simulink model "s_b4a4x4kf"  (R2018a)
settings: Solver=VariableStepDiscrete  StartTime=0.0  StopTime=1  RelTol=1e-3
undefined symbols (not defined in the file): fft_stages, n_bits_ants, n_bits_xengs
libraries: xbsIndex_r4 x22457, casper_library_misc x31, xbsReplacements_r4 x30, casper_library_scopes x17, xps_library x4
(part 155 of 232)

== system s_b4a4x4kf/sys0/vacc/vacc_time/snap/buscreate ==
  in1 : Inport
  in2 : Inport  Port=2
  in3 : Inport  Port=3
  in4 : Inport  Port=4
  in5 : Inport  Port=5
  in6 : Inport  Port=6
  in7 : Inport  Port=7
  in8 : Inport  Port=8
  in9 : Inport  Port=9
  in10 : Inport  Port=10
  concatenate : xbsIndex_r4/Concat  num_inputs=10  dbl_ovrd=off  block_type=concat
  reinterpret{1..10} (10 alike) : xbsIndex_r4/Reinterpret  force_arith_type=on  arith_type=Unsigned  force_bin_pt=on  bin_pt=0  block_type=reinterpret
      reinterpret1 settings: infoedit="Changes signal type without altering the binary representation.   You can changed the signal between signed and unsigned, and relocate the binary point.<br><br>Hardware notes: In hardware this block costs nothing.<br><br>Example:  Suppose the input is 6 bits wide, signed, with 2 fractional bits, and the output is forced to unsigned with 0 fractional bits.  Then an input of -2.0 (1110.00 in binary 2's complement) becomes an output of 56 (111000 in binary)."
      reinterpret2 settings: infoedit="Changes signal type without altering the binary representation.   You can changed the signal between signed and unsigned, and relocate the binary point.<br><br>Hardware notes: In hardware this block costs nothing.<br><br>Example:  Suppose the input is 6 bits wide, signed, with 2 fractional bits, and the output is forced to unsigned with 0 fractional bits.  Then an input of -2.0 (1110.00 in binary 2's complement) becomes an output of 56 (111000 in binary)."
  bus_out : Outport
  wires:
  concatenate/1 -> bus_out/1
  in1/1 -> reinterpret1/1
  reinterpret1/1 -> concatenate/1
  in2/1 -> reinterpret2/1
  reinterpret2/1 -> concatenate/2
  in3/1 -> reinterpret3/1
  reinterpret3/1 -> concatenate/3
  in4/1 -> reinterpret4/1
  reinterpret4/1 -> concatenate/4
  in5/1 -> reinterpret5/1
  reinterpret5/1 -> concatenate/5
  in6/1 -> reinterpret6/1
  reinterpret6/1 -> concatenate/6
  in7/1 -> reinterpret7/1
  reinterpret7/1 -> concatenate/7
  in8/1 -> reinterpret8/1
  reinterpret8/1 -> concatenate/8
  in9/1 -> reinterpret9/1
  reinterpret9/1 -> concatenate/9
  in10/1 -> reinterpret10/1
  reinterpret10/1 -> concatenate/10

== system s_b4a4x4kf/sys0/vacc/vacc_time/snap/io_delay ==
  d : Inport
  Register0 : xbsIndex_r4/Register  init=0  rst=off  en=off  dbl_ovrd=off  block_type=register
      settings: block_version=11.4
  Register1 : xbsIndex_r4/Register  init=0  rst=off  en=off  dbl_ovrd=off  block_type=register
      settings: block_version=11.4
  q : Outport
  wires:
  Register1/1 -> q/1
  d/1 -> Register0/1
  Register0/1 -> Register1/1

== system s_b4a4x4kf/sys0/vacc/vacc_time/snap/ss ==
  note: Generate stop
      | when in circular
      | capture mode
  note: Delay start
      | of capture
  note: ctrl:
      | bit0: Put a posedge here
      |         to enable a new capture.
      | bit1: ignore external trigger
      |         and trigger immediately.
      | bit2: ignore external write
      |         enable and capture on
      |         every FPGA clock.
      | bit3: continuously capture
      |         data until we get an
      |         external stop command.
  note: Offset in vector
      | from first element
      | captured, used
      | during circular capture
  note: Number of
      | bytes in
      | buffer and
      | done bit
  note: Number of valid
      | data samples to
      | skip after trigger
      | before starting
      | capture
  note: Value on vin
      | aligned with
      | first sample on
      | din captured
  din : Inport
  we : Inport  Port=2
  trig : Inport  Port=3
  stop : Inport  Port=4
  add_del : xbsIndex_r4/Delay  rst=off  infoeditControl=Selection of Reset will increase slice count due to use of real FFs and instead of SRLs  en=off  latency=1  reg_retiming=on  dbl_ovrd=off  block_type=delay
      settings: block_version=11.4
  add_gen : Subsystem  AncestorBlock=casper_library_scopes/snapshot/add_gen  mask{counter_size=32, increment=8, nsamples=11, burst_size=0, use_dsp48=on}
      mask prompts: counter_size "Address counter size (2^?)"; increment "Address counter increment"; nsamples "Number of samples (2^?)"; burst_size "Burst size (2^?)"; use_dsp48 "dsp48 counter/s"
      mask init:
      | set_param(gcb,'LinkStatus','inactive');
      | if strcmp(use_dsp48,'on'),
      |     set_param([gcb,'/add_gen'],'implementation','DSP48');
      | else
      |     set_param([gcb,'/add_gen'],'implementation','Fabric');
      | end
  arm : xbsIndex_r4/Constant  const=0  gui_display_data_type=Fixed-point  arith_type=Boolean  n_bits=16  bin_pt=14  preci_type=Single  exp_width=8  frac_width=24  explicit_period=on  period=1  equ=P=C  opselect=C  inp2=PCIN>>17  opr=+  inp1=P  carry=CIN  dbl_ovrd=off  block_type=constant
  arm_or : xbsIndex_r4/Logical  logical_function=OR  inputs=2  en=off  latency=0  precision=Full  arith_type=Unsigned  n_bits=16  bin_pt=0  align_bp=on  dbl_ovrd=off  block_type=logical
  basic_ctrl : Subsystem  AncestorBlock=casper_library_scopes/snapshot/basic_ctrl  mask{dram=off, data_width=64}
      mask prompts: data_width "data width"
      mask init:
      | set_param(gcb,'LinkStatus','inactive');
      | set_param([gcb,'/dram_munge'], 'dram', dram);
  bram : Subsystem  Tag=xps:bram  AncestorBlock=xps_library/Memory/shared_bram  mask{arith_type=Unsigned, addr_width=11, data_width=64, reg_prim_output=off, reg_core_output=off, optimization=Minimum_Area, data_bin_pt=0, init_vals=[0:2^11-1], sample_rate=1}
      mask prompts: arith_type "Output Data Type"; addr_width "Address width"; data_width "Data Width"; reg_prim_output "Register Primitive Output"; reg_core_output "Register Core Output"; data_bin_pt "Data Binary Point"; init_vals "Initial values (simulation only)"; sample_rate "Sample rate"
      mask init:
      | shared_bram_mask;
      mask TypeOptions arith_type: Unsigned | Signed  (2's comp)
      mask TypeOptions data_width: 8 | 16 | 32 | 64 | 128
      mask TypeOptions optimization: Minimum_Area | Low_Power
  cast : xbsIndex_r4/Convert  gui_display_data_type=Fixed-point  arith_type=Unsigned  n_bits=64  bin_pt=0  float_type=Single  exp_bits=8  fraction_bits=24  quantization=Truncate  overflow=Wrap  en=off  latency=0  pipeline=off  dbl_ovrd=off  block_type=convert
      settings: block_version=11.4
  circ : xbsIndex_r4/Constant  const=0  gui_display_data_type=Fixed-point  arith_type=Boolean  n_bits=16  bin_pt=14  preci_type=Single  exp_width=8  frac_width=24  explicit_period=on  period=1  equ=P=C  opselect=C  inp2=PCIN>>17  opr=+  inp1=P  carry=CIN  dbl_ovrd=off  block_type=constant
  circ_or : xbsIndex_r4/Logical  logical_function=OR  inputs=2  en=off  latency=0  precision=Full  arith_type=Unsigned  n_bits=16  bin_pt=0  align_bp=on  dbl_ovrd=off  block_type=logical
  ctrl : Subsystem  Tag=xps:sw_reg  AncestorBlock=xps_library/Memory/software_register  mask(swreg){io_dir=From Processor, io_delay=0, init_val=0, sample_period=1, names=reg, bitwidths=32, bin_pts=0, arith_types=0, sim_port=off, show_format=on}
      mask prompts: io_dir "I/O direction"; io_delay "I/O delay"; init_val "Initial Value"; sample_period "Sample period"; names "Bitfield names [msb...lsb]"; bitwidths "Bitfield widths"; bin_pts "Bitfield binary pts"; arith_types "Bitfield types, ufix=0, fix=1, bool=2"; sim_port "Provide sim input/output?"; show_format "Print format string?"
      mask help: A 32-bit software-accessible register. Can be divided into bitfields of varying widths and types using the fields in the block mask.
      mask init:
      | swreg_init(gcb)
      settings: AttributesFormatString=1input:uf32.0 = 32 bits
      mask TypeOptions io_dir: To Processor | From Processor
      mask Callback io_dir:
      | mask_enables = get_param(gcb, 'MaskEnables');
      | mask_names = get_param(gcb, 'MaskNames');
      | if strcmp(get_param(gcb, 'io_dir'), 'To Processor'),
      |     mask_enables{ismember(mask_names, 'sample_period')} = 'off';
      | else
      |     mask_enables{ismember(mask_names, 'sample_period')} = 'on';
      | end
      | set_param(gcb, 'MaskEnables', mask_enables);
      mask DialogControl ParameterTabVar0 Prompt: Setup
  ctrl_combine : Subsystem  AncestorBlock=casper_library_flow_control/bus_create  mask(bus_create){inputNum=4}
      mask prompts: inputNum "Number of inputs:"
      mask init:
      | bus_create_init(gcb,...
      |     'inputNum', inputNum);
  ctrl_split : Subsystem  AncestorBlock=casper_library_flow_control/bus_expand  mask(bus_expand){mode=divisions of arbitrary size, outputNum=1, outputWidth=[28 1 2 1], outputBinaryPt=0, outputArithmeticType=[0 2 0 2], show_format=on, outputToWorkspace=off, variablePrefix=out, outputToModelAsWell=on}
      mask prompts: outputNum "Number of outputs:"; outputWidth "Output width [msb ... lsb]:"; outputBinaryPt "Output binary point position [msb ... lsb]:"; outputArithmeticType "Output arithmetic type (ufix=0, fix=1, bool=2) [msb ... lsb]:"; show_format "Print format string?"; outputToWorkspace "Output to workspace?"; variablePrefix "Variable name prefix:"; outputToModelAsWell "Output to model as well?"
      mask help:
      | Expands a 'bus' made using a bus_create or Xilinx
      | concat block.
      | The input will be divided into the specified number
      | of outputs with the specified arithmetic types.
      | Divisions are made from most significant bit.
      mask init: same as s_b4a4x4kf/bus_expand
      settings: AttributesFormatString=4 outputs: uf28.0,b,uf2.0,b,
      mask TypeOptions mode: divisions of equal size | divisions of arbitrary size
      mask Callback mode: bus_expand_callback();
      mask Callback outputWidth: bus_expand_callback();
      mask Callback outputToWorkspace: bus_expand_callback();
  dat_del : xbsIndex_r4/Delay  rst=off  infoeditControl=Selection of Reset will increase slice count due to use of real FFs and instead of SRLs  en=off  latency=1  reg_retiming=on  dbl_ovrd=off  block_type=delay
      settings: block_version=11.4
  gbram : Terminator
  goto_ss_we2_const : xbsIndex_r4/Constant  const=0  gui_display_data_type=Fixed-point  arith_type=Boolean  n_bits=16  bin_pt=14  preci_type=Single  exp_width=8  frac_width=24  explicit_period=on  period=1  equ=P=C  opselect=C  inp2=PCIN>>17  opr=+  inp1=P  carry=CIN  dbl_ovrd=off  block_type=constant
  gval : Terminator
  ri : xbsIndex_r4/Reinterpret  force_arith_type=on  arith_type=Unsigned  force_bin_pt=on  bin_pt=0  block_type=reinterpret
      settings: infoedit="Changes signal type without altering the binary representation.   You can changed the signal between signed and unsigned, and relocate the binary point.<br><br>Hardware notes: In hardware this block costs nothing.<br><br>Example:  Suppose the input is 6 bits wide, signed, with 2 fractional bits, and the output is forced to unsigned with 0 fractional bits.  Then an input of -2.0 (1110.00 in binary 2's complement) becomes an output of 56 (111000 in binary)."
  status : Subsystem  Tag=xps:sw_reg  AncestorBlock=xps_library/Memory/software_register  mask(swreg){io_dir=To Processor, io_delay=0, init_val=0, sample_period=1, names=reg, bitwidths=32, bin_pts=0, arith_types=0, sim_port=off, show_format=on}
      mask prompts: io_dir "I/O direction"; io_delay "I/O delay"; init_val "Initial Value"; sample_period "Sample period"; names "Bitfield names [msb...lsb]"; bitwidths "Bitfield widths"; bin_pts "Bitfield binary pts"; arith_types "Bitfield types, ufix=0, fix=1, bool=2"; sim_port "Provide sim input/output?"; show_format "Print format string?"
      mask help: A 32-bit software-accessible register. Can be divided into bitfields of varying widths and types using the fields in the block mask.
      mask init:
      | swreg_init(gcb)
      settings: AttributesFormatString=1output:uf32.0 = 32 bits
      mask TypeOptions io_dir: To Processor | From Processor
      mask Callback io_dir:
      | mask_enables = get_param(gcb, 'MaskEnables');
      | mask_names = get_param(gcb, 'MaskNames');
      | if strcmp(get_param(gcb, 'io_dir'), 'To Processor'),
      |     mask_enables{ismember(mask_names, 'sample_period')} = 'off';
      | else
      |     mask_enables{ismember(mask_names, 'sample_period')} = 'on';
      | end
      | set_param(gcb, 'MaskEnables', mask_enables);
      mask DialogControl ParameterTabVar0 Prompt: Setup
  stop_gen : casper_library_scopes/snapshot/stop_gen
      settings: SourceProductName=CASPER DSP Blockset
  tr_en_cnt : Subsystem  Tag=xps:sw_reg  AncestorBlock=xps_library/Memory/software_register  mask(swreg){io_dir=To Processor, io_delay=0, init_val=0, sample_period=1, names=reg, bitwidths=32, bin_pts=0, arith_types=0, sim_port=off, show_format=on}
      mask prompts: io_dir "I/O direction"; io_delay "I/O delay"; init_val "Initial Value"; sample_period "Sample period"; names "Bitfield names [msb...lsb]"; bitwidths "Bitfield widths"; bin_pts "Bitfield binary pts"; arith_types "Bitfield types, ufix=0, fix=1, bool=2"; sim_port "Provide sim input/output?"; show_format "Print format string?"
      mask help: A 32-bit software-accessible register. Can be divided into bitfields of varying widths and types using the fields in the block mask.
      mask init:
      | swreg_init(gcb)
      settings: AttributesFormatString=1output:uf32.0 = 32 bits
      mask TypeOptions io_dir: To Processor | From Processor
      mask Callback io_dir:
      | mask_enables = get_param(gcb, 'MaskEnables');
      | mask_names = get_param(gcb, 'MaskNames');
      | if strcmp(get_param(gcb, 'io_dir'), 'To Processor'),
      |     mask_enables{ismember(mask_names, 'sample_period')} = 'off';
      | else
      |     mask_enables{ismember(mask_names, 'sample_period')} = 'on';
      | end
      | set_param(gcb, 'MaskEnables', mask_enables);
      mask DialogControl ParameterTabVar0 Prompt: Setup
  vin_const : xbsIndex_r4/Constant  const=0  gui_display_data_type=Fixed-point  arith_type=Boolean  n_bits=16  bin_pt=14  preci_type=Single  exp_width=8  frac_width=24  explicit_period=on  period=1  equ=P=C  opselect=C  inp2=PCIN>>17  opr=+  inp1=P  carry=CIN  dbl_ovrd=off  block_type=constant
  we_del : xbsIndex_r4/Delay  rst=off  infoeditControl=Selection of Reset will increase slice count due to use of real FFs and instead of SRLs  en=off  latency=1  reg_retiming=on  dbl_ovrd=off  block_type=delay
      settings: block_version=11.4
  arm_out : Outport
  tag scope: goto_98869994_we1=global, goto_98869994_we2=global, goto_98869994_we3=global, goto_98869994_we4=global
  wires:
  din/1 -> ri/1
  ri/1 -> cast/1
  cast/1 -> basic_ctrl/2(din)
  we/1 -> basic_ctrl/3(we)
  trig/1 -> basic_ctrl/4(trig)
  ctrl_combine/1(bus_out) -> basic_ctrl/5(ctrl), stop_gen/7
  stop/1 -> basic_ctrl/6(stopi)
  arm/1 -> arm_or/2
  arm_or/1 -> arm_out/1, ctrl_combine/4(in4)
  circ/1 -> circ_or/2
  ctrl/1(in_reg) -> ctrl_split/1(bus_in)
  ctrl_split/1(msb_out4) -> ctrl_combine/1(in1)
  ctrl_split/2(out3) -> circ_or/1
  ctrl_split/3(out2) -> ctrl_combine/3(in3)
  ctrl_split/4(lsb_out1) -> arm_or/1
  circ_or/1 -> ctrl_combine/2(in2)
  basic_ctrl/1(vout) -> stop_gen/1
  basic_ctrl/2(dout) -> stop_gen/2
  basic_ctrl/3(we_o) -> stop_gen/3, [goto_98869994_we1]
  basic_ctrl/4(go) -> stop_gen/4
  basic_ctrl/5(stop) -> stop_gen/5
  basic_ctrl/6(init) -> stop_gen/6
  stop_gen/1 -> add_gen/1(vin)
  stop_gen/2 -> add_gen/2(din)
  stop_gen/3 -> add_gen/3(we), [goto_98869994_we3]
  stop_gen/4 -> add_gen/4(go)
  stop_gen/5 -> add_gen/5(cont)
  stop_gen/6 -> add_gen/6(init)
  add_gen/5(status) -> status/1(out_reg)
  vin_const/1 -> basic_ctrl/1(vin)
  add_gen/1(vout) -> gval/1
  add_gen/6(en_cnt) -> tr_en_cnt/1(out_reg)
  add_gen/2(add) -> add_del/1
  add_gen/3(dout) -> dat_del/1
  add_gen/4(we_o) -> we_del/1, [goto_98869994_we4]
  add_del/1 -> bram/1(addr)
  dat_del/1 -> bram/2(data_in)
  we_del/1 -> bram/3(we)
  bram/1(data_out) -> gbram/1
  goto_ss_we2_const/1 -> [goto_98869994_we2]

== system s_b4a4x4kf/sys0/vacc/vacc_time/snap/stop_delay ==
  d : Inport
  Register0 : xbsIndex_r4/Register  init=0  rst=off  en=off  dbl_ovrd=off  block_type=register
      settings: block_version=11.4
  Register1 : xbsIndex_r4/Register  init=0  rst=off  en=off  dbl_ovrd=off  block_type=register
      settings: block_version=11.4
  q : Outport
  wires:
  Register1/1 -> q/1
  d/1 -> Register0/1
  Register0/1 -> Register1/1

== system s_b4a4x4kf/sys0/vacc/vacc_time/snap/trig_delay ==
  d : Inport
  Register0 : xbsIndex_r4/Register  init=0  rst=off  en=off  dbl_ovrd=off  block_type=register
      settings: block_version=11.4
  Register1 : xbsIndex_r4/Register  init=0  rst=off  en=off  dbl_ovrd=off  block_type=register
      settings: block_version=11.4
  q : Outport
  wires:
  Register1/1 -> q/1
  d/1 -> Register0/1
  Register0/1 -> Register1/1

== system s_b4a4x4kf/sys0/vacc/vacc_time/snap/we_delay ==
  d : Inport
  Register0 : xbsIndex_r4/Register  init=0  rst=off  en=off  dbl_ovrd=off  block_type=register
      settings: block_version=11.4
  Register1 : xbsIndex_r4/Register  init=0  rst=off  en=off  dbl_ovrd=off  block_type=register
      settings: block_version=11.4
  q : Outport
  wires:
  Register1/1 -> q/1
  d/1 -> Register0/1
  Register0/1 -> Register1/1

== system s_b4a4x4kf/sys0/vacc_tvg0/generate_time/segment/edge_detect ==
  in : Inport
  Delay : xbsIndex_r4/Delay  rst=off  infoeditControl=Selection of Reset will increase slice count due to use of real FFs and instead of SRLs  en=off  latency=1  reg_retiming=off  dbl_ovrd=off  block_type=delay
      settings: xl_area=[0, 0, 0, 0, 0, 0, 0]
  Inverter : xbsIndex_r4/Inverter  en=off  latency=0  dbl_ovrd=off  block_type=inv
      settings: xl_area=[0, 0, 0, 0, 0, 0, 0]
  edge_op : xbsIndex_r4/Logical  logical_function=NOR  inputs=2  en=off  latency=0  precision=Full  arith_type=Unsigned  n_bits=8  bin_pt=2  align_bp=on  dbl_ovrd=off  block_type=logical
      settings: xl_area=[0, 0, 0, 0, 0, 0, 0]
  out : Outport
  wires:
  Inverter/1 -> edge_op/1
  edge_op/1 -> out/1
  in/1 -> Inverter/1, Delay/1
  Delay/1 -> edge_op/2

== system s_b4a4x4kf/sys0/vacc_tvg0/ins_counter/bus_replicate1/bussify ==
  in1 : Inport
  in2 : Inport  Port=2
  in3 : Inport  Port=3
  in4 : Inport  Port=4
  in5 : Inport  Port=5
  in6 : Inport  Port=6
  in7 : Inport  Port=7
  in8 : Inport  Port=8
  concatenate : xbsIndex_r4/Concat  num_inputs=8  dbl_ovrd=off  block_type=concat
  reinterpret{1..8} (8 alike) : xbsIndex_r4/Reinterpret  force_arith_type=on  arith_type=Unsigned  force_bin_pt=on  bin_pt=0  block_type=reinterpret
      reinterpret1 settings: infoedit="Changes signal type without altering the binary representation.   You can changed the signal between signed and unsigned, and relocate the binary point.<br><br>Hardware notes: In hardware this block costs nothing.<br><br>Example:  Suppose the input is 6 bits wide, signed, with 2 fractional bits, and the output is forced to unsigned with 0 fractional bits.  Then an input of -2.0 (1110.00 in binary 2's complement) becomes an output of 56 (111000 in binary)."
      reinterpret2 settings: infoedit="Changes signal type without altering the binary representation.   You can changed the signal between signed and unsigned, and relocate the binary point.<br><br>Hardware notes: In hardware this block costs nothing.<br><br>Example:  Suppose the input is 6 bits wide, signed, with 2 fractional bits, and the output is forced to unsigned with 0 fractional bits.  Then an input of -2.0 (1110.00 in binary 2's complement) becomes an output of 56 (111000 in binary)."
  bus_out : Outport
  wires:
  concatenate/1 -> bus_out/1
  in1/1 -> reinterpret1/1
  reinterpret1/1 -> concatenate/1
  in2/1 -> reinterpret2/1
  reinterpret2/1 -> concatenate/2
  in3/1 -> reinterpret3/1
  reinterpret3/1 -> concatenate/3
  in4/1 -> reinterpret4/1
  reinterpret4/1 -> concatenate/4
  in5/1 -> reinterpret5/1
  reinterpret5/1 -> concatenate/5
  in6/1 -> reinterpret6/1
  reinterpret6/1 -> concatenate/6
  in7/1 -> reinterpret7/1
  reinterpret7/1 -> concatenate/7
  in8/1 -> reinterpret8/1
  reinterpret8/1 -> concatenate/8

== system s_b4a4x4kf/sys0/vacc_tvg0/ins_counter2/bus_replicate1/bussify ==
  in1 : Inport
  in2 : Inport  Port=2
  in3 : Inport  Port=3
  in4 : Inport  Port=4
  in5 : Inport  Port=5
  in6 : Inport  Port=6
  in7 : Inport  Port=7
  in8 : Inport  Port=8
  concatenate : xbsIndex_r4/Concat  num_inputs=8  dbl_ovrd=off  block_type=concat
  reinterpret{1..8} (8 alike) : xbsIndex_r4/Reinterpret  force_arith_type=on  arith_type=Unsigned  force_bin_pt=on  bin_pt=0  block_type=reinterpret
      reinterpret1 settings: infoedit="Changes signal type without altering the binary representation.   You can changed the signal between signed and unsigned, and relocate the binary point.<br><br>Hardware notes: In hardware this block costs nothing.<br><br>Example:  Suppose the input is 6 bits wide, signed, with 2 fractional bits, and the output is forced to unsigned with 0 fractional bits.  Then an input of -2.0 (1110.00 in binary 2's complement) becomes an output of 56 (111000 in binary)."
      reinterpret2 settings: infoedit="Changes signal type without altering the binary representation.   You can changed the signal between signed and unsigned, and relocate the binary point.<br><br>Hardware notes: In hardware this block costs nothing.<br><br>Example:  Suppose the input is 6 bits wide, signed, with 2 fractional bits, and the output is forced to unsigned with 0 fractional bits.  Then an input of -2.0 (1110.00 in binary 2's complement) becomes an output of 56 (111000 in binary)."
  bus_out : Outport
  wires:
  concatenate/1 -> bus_out/1
  in1/1 -> reinterpret1/1
  reinterpret1/1 -> concatenate/1
  in2/1 -> reinterpret2/1
  reinterpret2/1 -> concatenate/2
  in3/1 -> reinterpret3/1
  reinterpret3/1 -> concatenate/3
  in4/1 -> reinterpret4/1
  reinterpret4/1 -> concatenate/4
  in5/1 -> reinterpret5/1
  reinterpret5/1 -> concatenate/5
  in6/1 -> reinterpret6/1
  reinterpret6/1 -> concatenate/6
  in7/1 -> reinterpret7/1
  reinterpret7/1 -> concatenate/7
  in8/1 -> reinterpret8/1
  reinterpret8/1 -> concatenate/8

== system s_b4a4x4kf/sys0/vacc_tvg0/ins_counter2/segment/edge_detect ==
  in : Inport
  Delay : xbsIndex_r4/Delay  rst=off  infoeditControl=Selection of Reset will increase slice count due to use of real FFs and instead of SRLs  en=off  latency=1  reg_retiming=off  dbl_ovrd=off  block_type=delay
      settings: xl_area=[0, 0, 0, 0, 0, 0, 0]
  Inverter : xbsIndex_r4/Inverter  en=off  latency=0  dbl_ovrd=off  block_type=inv
      settings: xl_area=[0, 0, 0, 0, 0, 0, 0]
  edge_op : xbsIndex_r4/Logical  logical_function=NOR  inputs=2  en=off  latency=0  precision=Full  arith_type=Unsigned  n_bits=8  bin_pt=2  align_bp=on  dbl_ovrd=off  block_type=logical
      settings: xl_area=[0, 0, 0, 0, 0, 0, 0]
  out : Outport
  wires:
  Inverter/1 -> edge_op/1
  edge_op/1 -> out/1
  in/1 -> Inverter/1, Delay/1
  Delay/1 -> edge_op/2

== system s_b4a4x4kf/sys0/vacc_tvg0/ins_counter3/bus_replicate1/bussify ==
  in1 : Inport
  in2 : Inport  Port=2
  in3 : Inport  Port=3
  in4 : Inport  Port=4
  in5 : Inport  Port=5
  in6 : Inport  Port=6
  in7 : Inport  Port=7
  in8 : Inport  Port=8
  concatenate : xbsIndex_r4/Concat  num_inputs=8  dbl_ovrd=off  block_type=concat
  reinterpret{1..8} (8 alike) : xbsIndex_r4/Reinterpret  force_arith_type=on  arith_type=Unsigned  force_bin_pt=on  bin_pt=0  block_type=reinterpret
      reinterpret1 settings: infoedit="Changes signal type without altering the binary representation.   You can changed the signal between signed and unsigned, and relocate the binary point.<br><br>Hardware notes: In hardware this block costs nothing.<br><br>Example:  Suppose the input is 6 bits wide, signed, with 2 fractional bits, and the output is forced to unsigned with 0 fractional bits.  Then an input of -2.0 (1110.00 in binary 2's complement) becomes an output of 56 (111000 in binary)."
      reinterpret2 settings: infoedit="Changes signal type without altering the binary representation.   You can changed the signal between signed and unsigned, and relocate the binary point.<br><br>Hardware notes: In hardware this block costs nothing.<br><br>Example:  Suppose the input is 6 bits wide, signed, with 2 fractional bits, and the output is forced to unsigned with 0 fractional bits.  Then an input of -2.0 (1110.00 in binary 2's complement) becomes an output of 56 (111000 in binary)."
  bus_out : Outport
  wires:
  concatenate/1 -> bus_out/1
  in1/1 -> reinterpret1/1
  reinterpret1/1 -> concatenate/1
  in2/1 -> reinterpret2/1
  reinterpret2/1 -> concatenate/2
  in3/1 -> reinterpret3/1
  reinterpret3/1 -> concatenate/3
  in4/1 -> reinterpret4/1
  reinterpret4/1 -> concatenate/4
  in5/1 -> reinterpret5/1
  reinterpret5/1 -> concatenate/5
  in6/1 -> reinterpret6/1
  reinterpret6/1 -> concatenate/6
  in7/1 -> reinterpret7/1
  reinterpret7/1 -> concatenate/7
  in8/1 -> reinterpret8/1
  reinterpret8/1 -> concatenate/8

== system s_b4a4x4kf/sys0/vacc_tvg0/ins_counter3/segment/edge_detect ==
  in : Inport
  Delay : xbsIndex_r4/Delay  rst=off  infoeditControl=Selection of Reset will increase slice count due to use of real FFs and instead of SRLs  en=off  latency=1  reg_retiming=off  dbl_ovrd=off  block_type=delay
      settings: xl_area=[0, 0, 0, 0, 0, 0, 0]
  Inverter : xbsIndex_r4/Inverter  en=off  latency=0  dbl_ovrd=off  block_type=inv
      settings: xl_area=[0, 0, 0, 0, 0, 0, 0]
  edge_op : xbsIndex_r4/Logical  logical_function=NOR  inputs=2  en=off  latency=0  precision=Full  arith_type=Unsigned  n_bits=8  bin_pt=2  align_bp=on  dbl_ovrd=off  block_type=logical
      settings: xl_area=[0, 0, 0, 0, 0, 0, 0]
  out : Outport
  wires:
  Inverter/1 -> edge_op/1
  edge_op/1 -> out/1
  in/1 -> Inverter/1, Delay/1
  Delay/1 -> edge_op/2

== system s_b4a4x4kf/sys0/xeng/auto_tap/dual_pol_cmac/cmac1 ==
  a+bi : Inport
  c+di : Inport  Port=2
  acc_in : Inport  Port=3
  sync : Inport  Port=4
  valid_in : Inport  Port=5
  Constant1 : xbsIndex_r4/Constant  const=0  gui_display_data_type=Fixed-point  arith_type=Unsigned  n_bits=bit_growth  bin_pt=0  preci_type=Single  exp_width=8  frac_width=24  explicit_period=on  period=1  equ=P=C  opselect=C  inp2=PCIN>>17  opr=+  inp1=P  carry=CIN  dbl_ovrd=off  block_type=constant
      settings: block_version=9.2.01
  Constant2 : xbsIndex_r4/Constant  const=0  gui_display_data_type=Fixed-point  arith_type=Unsigned  n_bits=1  bin_pt=0  preci_type=Single  exp_width=8  frac_width=24  explicit_period=off  period=1  equ=P=C  opselect=C  inp2=PCIN>>17  opr=+  inp1=P  carry=CIN  dbl_ovrd=off  block_type=constant
      settings: block_version=9.2.01
  Counter : xbsIndex_r4/Counter  cnt_type=Count Limited  cnt_to=acc_len - 1  operation=Up  start_count=0  cnt_by_val=1  arith_type=Unsigned  n_bits=bit_growth  bin_pt=0  load_pin=off  rst=on  en=off  explicit_period=off  period=1  use_behavioral_HDL=off  implementation=Fabric  use_rpm=on  dbl_ovrd=off  block_type=counter
      settings: xl_area=[0, 0, 0, 0, 0, 0, 0]  block_version=9.2.01
  Delay : xbsIndex_r4/Delay  rst=off  infoeditControl=Selection of Reset will increase slice count due to use of real FFs and instead of SRLs  en=off  latency=add_latency + mult_latency - 1  reg_retiming=on  dbl_ovrd=off  block_type=delay
      settings: xl_area=[0, 0, 0, 0, 0, 0, 0]  block_version=9.2.01
  Relational : xbsIndex_r4/Relational  mode=a=b  op_type=Bool  en=off  latency=1  dbl_ovrd=off  block_type=relational
      settings: xl_area=[0, 0, 0, 0, 0, 0, 0]  block_version=9.2.01
  Terminator : Terminator
  acc : Subsystem
  acc1 : Subsystem
  c_to_ri1 : Subsystem
  c_to_ri2 : Subsystem
  cmult* : Subsystem  mask(cmult){n_bits_a=8, bin_pt_a=7, n_bits_b=8, bin_pt_b=7, n_bits_ab=25, bin_pt_ab=14, quantization=Truncate, overflow=Wrap, in_latency=0, mult_latency=4, add_latency=3, conv_latency=0, conjugated=on, async=off, pipelined_enable=on, multiplier_implementation=embedded multiplier core}
      mask prompts: n_bits_a "Number of Bits 'a'"; bin_pt_a "Binary Point 'a'"; n_bits_b "Number of Bits 'b'"; bin_pt_b "Binary Point 'b'"; n_bits_ab "Number of Bits 'ab'"; bin_pt_ab "Binary Point 'ab'"; in_latency "Input latency"; mult_latency "Multiplier Latency"; add_latency "Adder Latency"; conv_latency "Convert latency"; conjugated "Conjugate"; async "asynchronous operation"; pipelined_enable "enable pipeline"; multiplier_implementation "Multiplier implementation"
      mask help:
      | Multiplies two complex numbers using 4 multipliers and 2 adders.
      | Conjugation is optional.
      mask init:
      | cmult_init(gcb, ...
      |     'n_bits_a',n_bits_a, ...
      |     'bin_pt_a',bin_pt_a, ...
      |     'n_bits_b',n_bits_b, ...
      |     'bin_pt_b',bin_pt_b, ...
      |     'n_bits_ab',n_bits_ab, ...
      |     'bin_pt_ab',bin_pt_ab, ...
      |     'quantization',quantization, ...
      |     'overflow', overflow, ...
      |     'in_latency', in_latency, ...
      |     'mult_latency', mult_latency, ...
      |     'add_latency', add_latency, ...
      |     'conv_latency', conv_latency, ...
      |     'conjugated', conjugated, ...
      |     'multiplier_implementation', multiplier_implementation, ...
      |     'async', async, ...
      |     'pipelined_enable', pipelined_enable);
      settings: AttributesFormatString=|
      | 8_7 * 8_7 ==> 25_14
      | Truncate, Wrap
      | Latency=0
      mask TypeOptions quantization: Truncate | Round  (unbiased: +/- Inf) | Round  (unbiased: Even Values)
      mask TypeOptions overflow: Wrap | Saturate | Flag as error
      mask TypeOptions multiplier_implementation: behavioral HDL | standard core | embedded multiplier core
  ri_to_c : Subsystem
  acc_out : Outport
  valid_out : Outport  Port=2
  wires:
  c_to_ri2/1(Out1) -> acc/3(acc_in)
  acc/1(acc_out) -> ri_to_c/1(In1)
  c_to_ri1/2(Out2) -> acc1/2(din)
  c_to_ri1/1(Out1) -> acc/2(din)  "auto_real"
  a+bi/1 -> cmult*/1(a)
  c+di/1 -> cmult*/2(b)
  acc_in/1 -> c_to_ri2/1(In1)
  acc1/1(acc_out) -> ri_to_c/2(In2)
  ri_to_c/1(Out1) -> acc_out/1
  c_to_ri2/2(Out2) -> acc1/3(acc_in)
  Relational/1 -> acc/1(rst), acc1/1(rst)
  Counter/1 -> Relational/1
  Constant1/1 -> Relational/2
  sync/1 -> Delay/1
  Delay/1 -> Counter/1
  Constant2/1 -> acc/4(valid_in)
  acc/2(valid_out) -> Terminator/1
  acc1/2(valid_out) -> valid_out/1
  valid_in/1 -> acc1/4(valid_in)
  cmult*/1(ab) -> c_to_ri1/1(In1)

== system s_b4a4x4kf/sys0/xeng/auto_tap/dual_pol_cmac/cmac2 ==
  a+bi : Inport
  c+di : Inport  Port=2
  acc_in : Inport  Port=3
  sync : Inport  Port=4
  valid_in : Inport  Port=5
  Constant1 : xbsIndex_r4/Constant  const=0  gui_display_data_type=Fixed-point  arith_type=Unsigned  n_bits=bit_growth  bin_pt=0  preci_type=Single  exp_width=8  frac_width=24  explicit_period=on  period=1  equ=P=C  opselect=C  inp2=PCIN>>17  opr=+  inp1=P  carry=CIN  dbl_ovrd=off  block_type=constant
      settings: block_version=9.2.01
  Constant2 : xbsIndex_r4/Constant  const=0  gui_display_data_type=Fixed-point  arith_type=Unsigned  n_bits=1  bin_pt=0  preci_type=Single  exp_width=8  frac_width=24  explicit_period=off  period=1  equ=P=C  opselect=C  inp2=PCIN>>17  opr=+  inp1=P  carry=CIN  dbl_ovrd=off  block_type=constant
      settings: block_version=9.2.01
  Counter : xbsIndex_r4/Counter  cnt_type=Count Limited  cnt_to=acc_len - 1  operation=Up  start_count=0  cnt_by_val=1  arith_type=Unsigned  n_bits=bit_growth  bin_pt=0  load_pin=off  rst=on  en=off  explicit_period=off  period=1  use_behavioral_HDL=off  implementation=Fabric  use_rpm=on  dbl_ovrd=off  block_type=counter
      settings: xl_area=[0, 0, 0, 0, 0, 0, 0]  block_version=9.2.01
  Delay : xbsIndex_r4/Delay  rst=off  infoeditControl=Selection of Reset will increase slice count due to use of real FFs and instead of SRLs  en=off  latency=add_latency + mult_latency - 1  reg_retiming=on  dbl_ovrd=off  block_type=delay
      settings: xl_area=[0, 0, 0, 0, 0, 0, 0]  block_version=9.2.01
  Relational : xbsIndex_r4/Relational  mode=a=b  op_type=Bool  en=off  latency=1  dbl_ovrd=off  block_type=relational
      settings: xl_area=[0, 0, 0, 0, 0, 0, 0]  block_version=9.2.01
  Terminator : Terminator
  acc : Subsystem
  acc1 : Subsystem
  c_to_ri1 : Subsystem
  c_to_ri2 : Subsystem
  cmult* : Subsystem  mask(cmult){n_bits_a=8, bin_pt_a=7, n_bits_b=8, bin_pt_b=7, n_bits_ab=25, bin_pt_ab=14, quantization=Truncate, overflow=Wrap, in_latency=0, mult_latency=4, add_latency=3, conv_latency=0, conjugated=on, async=off, pipelined_enable=on, multiplier_implementation=embedded multiplier core}
      mask prompts: n_bits_a "Number of Bits 'a'"; bin_pt_a "Binary Point 'a'"; n_bits_b "Number of Bits 'b'"; bin_pt_b "Binary Point 'b'"; n_bits_ab "Number of Bits 'ab'"; bin_pt_ab "Binary Point 'ab'"; in_latency "Input latency"; mult_latency "Multiplier Latency"; add_latency "Adder Latency"; conv_latency "Convert latency"; conjugated "Conjugate"; async "asynchronous operation"; pipelined_enable "enable pipeline"; multiplier_implementation "Multiplier implementation"
      mask help:
      | Multiplies two complex numbers using 4 multipliers and 2 adders.
      | Conjugation is optional.
      mask init: same as s_b4a4x4kf/sys0/xeng/auto_tap/dual_pol_cmac/cmac1/cmult*
      settings: AttributesFormatString=|
      | 8_7 * 8_7 ==> 25_14
      | Truncate, Wrap
      | Latency=0
      mask TypeOptions quantization: Truncate | Round  (unbiased: +/- Inf) | Round  (unbiased: Even Values)
      mask TypeOptions overflow: Wrap | Saturate | Flag as error
      mask TypeOptions multiplier_implementation: behavioral HDL | standard core | embedded multiplier core
  ri_to_c : Subsystem
  acc_out : Outport
  valid_out : Outport  Port=2
  wires:
  c_to_ri2/1(Out1) -> acc/3(acc_in)
  acc/1(acc_out) -> ri_to_c/1(In1)
  c_to_ri1/2(Out2) -> acc1/2(din)
  c_to_ri1/1(Out1) -> acc/2(din)  "auto_real"
  a+bi/1 -> cmult*/1(a)
  c+di/1 -> cmult*/2(b)
  acc_in/1 -> c_to_ri2/1(In1)
  acc1/1(acc_out) -> ri_to_c/2(In2)
  ri_to_c/1(Out1) -> acc_out/1
  c_to_ri2/2(Out2) -> acc1/3(acc_in)
  Relational/1 -> acc/1(rst), acc1/1(rst)
  Counter/1 -> Relational/1
  Constant1/1 -> Relational/2
  sync/1 -> Delay/1
  Delay/1 -> Counter/1
  Constant2/1 -> acc/4(valid_in)
  acc/2(valid_out) -> Terminator/1
  acc1/2(valid_out) -> valid_out/1
  valid_in/1 -> acc1/4(valid_in)
  cmult*/1(ab) -> c_to_ri1/1(In1)

== system s_b4a4x4kf/sys0/xeng/auto_tap/dual_pol_cmac/cmac3 ==
  a+bi : Inport
  c+di : Inport  Port=2
  acc_in : Inport  Port=3
  sync : Inport  Port=4
  valid_in : Inport  Port=5
  Constant1 : xbsIndex_r4/Constant  const=0  gui_display_data_type=Fixed-point  arith_type=Unsigned  n_bits=bit_growth  bin_pt=0  preci_type=Single  exp_width=8  frac_width=24  explicit_period=on  period=1  equ=P=C  opselect=C  inp2=PCIN>>17  opr=+  inp1=P  carry=CIN  dbl_ovrd=off  block_type=constant
      settings: block_version=9.2.01
  Constant2 : xbsIndex_r4/Constant  const=0  gui_display_data_type=Fixed-point  arith_type=Unsigned  n_bits=1  bin_pt=0  preci_type=Single  exp_width=8  frac_width=24  explicit_period=off  period=1  equ=P=C  opselect=C  inp2=PCIN>>17  opr=+  inp1=P  carry=CIN  dbl_ovrd=off  block_type=constant
      settings: block_version=9.2.01
  Counter : xbsIndex_r4/Counter  cnt_type=Count Limited  cnt_to=acc_len - 1  operation=Up  start_count=0  cnt_by_val=1  arith_type=Unsigned  n_bits=bit_growth  bin_pt=0  load_pin=off  rst=on  en=off  explicit_period=off  period=1  use_behavioral_HDL=off  implementation=Fabric  use_rpm=on  dbl_ovrd=off  block_type=counter
      settings: xl_area=[0, 0, 0, 0, 0, 0, 0]  block_version=9.2.01
  Delay : xbsIndex_r4/Delay  rst=off  infoeditControl=Selection of Reset will increase slice count due to use of real FFs and instead of SRLs  en=off  latency=add_latency + mult_latency - 1  reg_retiming=on  dbl_ovrd=off  block_type=delay
      settings: xl_area=[0, 0, 0, 0, 0, 0, 0]  block_version=9.2.01
  Relational : xbsIndex_r4/Relational  mode=a=b  op_type=Bool  en=off  latency=1  dbl_ovrd=off  block_type=relational
      settings: xl_area=[0, 0, 0, 0, 0, 0, 0]  block_version=9.2.01
  Terminator : Terminator
  acc : Subsystem
  acc1 : Subsystem
  c_to_ri1 : Subsystem
  c_to_ri2 : Subsystem
  cmult* : Subsystem  mask(cmult){n_bits_a=8, bin_pt_a=7, n_bits_b=8, bin_pt_b=7, n_bits_ab=25, bin_pt_ab=14, quantization=Truncate, overflow=Wrap, in_latency=0, mult_latency=4, add_latency=3, conv_latency=0, conjugated=on, async=off, pipelined_enable=on, multiplier_implementation=embedded multiplier core}
      mask prompts: n_bits_a "Number of Bits 'a'"; bin_pt_a "Binary Point 'a'"; n_bits_b "Number of Bits 'b'"; bin_pt_b "Binary Point 'b'"; n_bits_ab "Number of Bits 'ab'"; bin_pt_ab "Binary Point 'ab'"; in_latency "Input latency"; mult_latency "Multiplier Latency"; add_latency "Adder Latency"; conv_latency "Convert latency"; conjugated "Conjugate"; async "asynchronous operation"; pipelined_enable "enable pipeline"; multiplier_implementation "Multiplier implementation"
      mask help:
      | Multiplies two complex numbers using 4 multipliers and 2 adders.
      | Conjugation is optional.
      mask init: same as s_b4a4x4kf/sys0/xeng/auto_tap/dual_pol_cmac/cmac1/cmult*
      settings: AttributesFormatString=|
      | 8_7 * 8_7 ==> 25_14
      | Truncate, Wrap
      | Latency=0
      mask TypeOptions quantization: Truncate | Round  (unbiased: +/- Inf) | Round  (unbiased: Even Values)
      mask TypeOptions overflow: Wrap | Saturate | Flag as error
      mask TypeOptions multiplier_implementation: behavioral HDL | standard core | embedded multiplier core
  ri_to_c : Subsystem
  acc_out : Outport
  valid_out : Outport  Port=2
  wires:
  c_to_ri2/1(Out1) -> acc/3(acc_in)
  acc/1(acc_out) -> ri_to_c/1(In1)
  c_to_ri1/2(Out2) -> acc1/2(din)
  c_to_ri1/1(Out1) -> acc/2(din)  "auto_real"
  a+bi/1 -> cmult*/1(a)
  c+di/1 -> cmult*/2(b)
  acc_in/1 -> c_to_ri2/1(In1)
  acc1/1(acc_out) -> ri_to_c/2(In2)
  ri_to_c/1(Out1) -> acc_out/1
  c_to_ri2/2(Out2) -> acc1/3(acc_in)
  Relational/1 -> acc/1(rst), acc1/1(rst)
  Counter/1 -> Relational/1
  Constant1/1 -> Relational/2
  sync/1 -> Delay/1
  Delay/1 -> Counter/1
  Constant2/1 -> acc/4(valid_in)
  acc/2(valid_out) -> Terminator/1
  acc1/2(valid_out) -> valid_out/1
  valid_in/1 -> acc1/4(valid_in)
  cmult*/1(ab) -> c_to_ri1/1(In1)

== system s_b4a4x4kf/sys0/xeng/auto_tap/dual_pol_cmac/cmac4 ==
  a+bi : Inport
  c+di : Inport  Port=2
  acc_in : Inport  Port=3
  sync : Inport  Port=4
  valid_in : Inport  Port=5
  Constant1 : xbsIndex_r4/Constant  const=0  gui_display_data_type=Fixed-point  arith_type=Unsigned  n_bits=bit_growth  bin_pt=0  preci_type=Single  exp_width=8  frac_width=24  explicit_period=on  period=1  equ=P=C  opselect=C  inp2=PCIN>>17  opr=+  inp1=P  carry=CIN  dbl_ovrd=off  block_type=constant
      settings: block_version=9.2.01
  Constant2 : xbsIndex_r4/Constant  const=0  gui_display_data_type=Fixed-point  arith_type=Unsigned  n_bits=1  bin_pt=0  preci_type=Single  exp_width=8  frac_width=24  explicit_period=off  period=1  equ=P=C  opselect=C  inp2=PCIN>>17  opr=+  inp1=P  carry=CIN  dbl_ovrd=off  block_type=constant
      settings: block_version=9.2.01
  Counter : xbsIndex_r4/Counter  cnt_type=Count Limited  cnt_to=acc_len - 1  operation=Up  start_count=0  cnt_by_val=1  arith_type=Unsigned  n_bits=bit_growth  bin_pt=0  load_pin=off  rst=on  en=off  explicit_period=off  period=1  use_behavioral_HDL=off  implementation=Fabric  use_rpm=on  dbl_ovrd=off  block_type=counter
      settings: xl_area=[0, 0, 0, 0, 0, 0, 0]  block_version=9.2.01
  Delay : xbsIndex_r4/Delay  rst=off  infoeditControl=Selection of Reset will increase slice count due to use of real FFs and instead of SRLs  en=off  latency=add_latency + mult_latency - 1  reg_retiming=on  dbl_ovrd=off  block_type=delay
      settings: xl_area=[0, 0, 0, 0, 0, 0, 0]  block_version=9.2.01
  Relational : xbsIndex_r4/Relational  mode=a=b  op_type=Bool  en=off  latency=1  dbl_ovrd=off  block_type=relational
      settings: xl_area=[0, 0, 0, 0, 0, 0, 0]  block_version=9.2.01
  Terminator : Terminator
  acc : Subsystem
  acc1 : Subsystem
  c_to_ri1 : Subsystem
  c_to_ri2 : Subsystem
  cmult* : Subsystem  mask(cmult){n_bits_a=8, bin_pt_a=7, n_bits_b=8, bin_pt_b=7, n_bits_ab=25, bin_pt_ab=14, quantization=Truncate, overflow=Wrap, in_latency=0, mult_latency=4, add_latency=3, conv_latency=0, conjugated=on, async=off, pipelined_enable=on, multiplier_implementation=embedded multiplier core}
      mask prompts: n_bits_a "Number of Bits 'a'"; bin_pt_a "Binary Point 'a'"; n_bits_b "Number of Bits 'b'"; bin_pt_b "Binary Point 'b'"; n_bits_ab "Number of Bits 'ab'"; bin_pt_ab "Binary Point 'ab'"; in_latency "Input latency"; mult_latency "Multiplier Latency"; add_latency "Adder Latency"; conv_latency "Convert latency"; conjugated "Conjugate"; async "asynchronous operation"; pipelined_enable "enable pipeline"; multiplier_implementation "Multiplier implementation"
      mask help:
      | Multiplies two complex numbers using 4 multipliers and 2 adders.
      | Conjugation is optional.
      mask init: same as s_b4a4x4kf/sys0/xeng/auto_tap/dual_pol_cmac/cmac1/cmult*
      settings: AttributesFormatString=|
      | 8_7 * 8_7 ==> 25_14
      | Truncate, Wrap
      | Latency=0
      mask TypeOptions quantization: Truncate | Round  (unbiased: +/- Inf) | Round  (unbiased: Even Values)
      mask TypeOptions overflow: Wrap | Saturate | Flag as error
      mask TypeOptions multiplier_implementation: behavioral HDL | standard core | embedded multiplier core
  ri_to_c : Subsystem
  acc_out : Outport
  valid_out : Outport  Port=2
  wires:
  c_to_ri2/1(Out1) -> acc/3(acc_in)
  acc/1(acc_out) -> ri_to_c/1(In1)
  c_to_ri1/2(Out2) -> acc1/2(din)
  c_to_ri1/1(Out1) -> acc/2(din)  "auto_real"
  a+bi/1 -> cmult*/1(a)
  c+di/1 -> cmult*/2(b)
  acc_in/1 -> c_to_ri2/1(In1)
  acc1/1(acc_out) -> ri_to_c/2(In2)
  ri_to_c/1(Out1) -> acc_out/1
  c_to_ri2/2(Out2) -> acc1/3(acc_in)
  Relational/1 -> acc/1(rst), acc1/1(rst)
  Counter/1 -> Relational/1
  Constant1/1 -> Relational/2
  sync/1 -> Delay/1
  Delay/1 -> Counter/1
  Constant2/1 -> acc/4(valid_in)
  acc/2(valid_out) -> Terminator/1
  acc1/2(valid_out) -> valid_out/1
  valid_in/1 -> acc1/4(valid_in)
  cmult*/1(ab) -> c_to_ri1/1(In1)

== system s_b4a4x4kf/sys0/xeng/baseline_tap1/dual_pol_cmac/cmac1 ==
  a+bi : Inport
  c+di : Inport  Port=2
  acc_in : Inport  Port=3
  sync : Inport  Port=4
  valid_in : Inport  Port=5
  Constant1 : xbsIndex_r4/Constant  const=0  gui_display_data_type=Fixed-point  arith_type=Unsigned  n_bits=bit_growth  bin_pt=0  preci_type=Single  exp_width=8  frac_width=24  explicit_period=on  period=1  equ=P=C  opselect=C  inp2=PCIN>>17  opr=+  inp1=P  carry=CIN  dbl_ovrd=off  block_type=constant
      settings: block_version=9.2.01
  Constant2 : xbsIndex_r4/Constant  const=0  gui_display_data_type=Fixed-point  arith_type=Unsigned  n_bits=1  bin_pt=0  preci_type=Single  exp_width=8  frac_width=24  explicit_period=off  period=1  equ=P=C  opselect=C  inp2=PCIN>>17  opr=+  inp1=P  carry=CIN  dbl_ovrd=off  block_type=constant
      settings: block_version=9.2.01
  Counter : xbsIndex_r4/Counter  cnt_type=Count Limited  cnt_to=acc_len - 1  operation=Up  start_count=0  cnt_by_val=1  arith_type=Unsigned  n_bits=bit_growth  bin_pt=0  load_pin=off  rst=on  en=off  explicit_period=off  period=1  use_behavioral_HDL=off  implementation=Fabric  use_rpm=on  dbl_ovrd=off  block_type=counter
      settings: xl_area=[0, 0, 0, 0, 0, 0, 0]  block_version=9.2.01
  Delay : xbsIndex_r4/Delay  rst=off  infoeditControl=Selection of Reset will increase slice count due to use of real FFs and instead of SRLs  en=off  latency=add_latency + mult_latency - 1  reg_retiming=on  dbl_ovrd=off  block_type=delay
      settings: xl_area=[0, 0, 0, 0, 0, 0, 0]  block_version=9.2.01
  Relational : xbsIndex_r4/Relational  mode=a=b  op_type=Bool  en=off  latency=1  dbl_ovrd=off  block_type=relational
      settings: xl_area=[0, 0, 0, 0, 0, 0, 0]  block_version=9.2.01
  Terminator : Terminator
  acc : Subsystem
  acc1 : Subsystem
  c_to_ri1 : Subsystem
  c_to_ri2 : Subsystem
  cmult* : Subsystem  mask(cmult){n_bits_a=8, bin_pt_a=7, n_bits_b=8, bin_pt_b=7, n_bits_ab=25, bin_pt_ab=14, quantization=Truncate, overflow=Wrap, in_latency=0, mult_latency=4, add_latency=3, conv_latency=0, conjugated=on, async=off, pipelined_enable=on, multiplier_implementation=embedded multiplier core}
      mask prompts: n_bits_a "Number of Bits 'a'"; bin_pt_a "Binary Point 'a'"; n_bits_b "Number of Bits 'b'"; bin_pt_b "Binary Point 'b'"; n_bits_ab "Number of Bits 'ab'"; bin_pt_ab "Binary Point 'ab'"; in_latency "Input latency"; mult_latency "Multiplier Latency"; add_latency "Adder Latency"; conv_latency "Convert latency"; conjugated "Conjugate"; async "asynchronous operation"; pipelined_enable "enable pipeline"; multiplier_implementation "Multiplier implementation"
      mask help:
      | Multiplies two complex numbers using 4 multipliers and 2 adders.
      | Conjugation is optional.
      mask init: same as s_b4a4x4kf/sys0/xeng/auto_tap/dual_pol_cmac/cmac1/cmult*
      settings: AttributesFormatString=|
      | 8_7 * 8_7 ==> 25_14
      | Truncate, Wrap
      | Latency=0
      mask TypeOptions quantization: Truncate | Round  (unbiased: +/- Inf) | Round  (unbiased: Even Values)
      mask TypeOptions overflow: Wrap | Saturate | Flag as error
      mask TypeOptions multiplier_implementation: behavioral HDL | standard core | embedded multiplier core
  ri_to_c : Subsystem
  acc_out : Outport
  valid_out : Outport  Port=2
  wires:
  c_to_ri2/1(Out1) -> acc/3(acc_in)
  acc/1(acc_out) -> ri_to_c/1(In1)
  c_to_ri1/2(Out2) -> acc1/2(din)
  c_to_ri1/1(Out1) -> acc/2(din)  "auto_real"
  a+bi/1 -> cmult*/1(a)
  c+di/1 -> cmult*/2(b)
  acc_in/1 -> c_to_ri2/1(In1)
  acc1/1(acc_out) -> ri_to_c/2(In2)
  ri_to_c/1(Out1) -> acc_out/1
  c_to_ri2/2(Out2) -> acc1/3(acc_in)
  Relational/1 -> acc/1(rst), acc1/1(rst)
  Counter/1 -> Relational/1
  Constant1/1 -> Relational/2
  sync/1 -> Delay/1
  Delay/1 -> Counter/1
  Constant2/1 -> acc/4(valid_in)
  acc/2(valid_out) -> Terminator/1
  acc1/2(valid_out) -> valid_out/1
  valid_in/1 -> acc1/4(valid_in)
  cmult*/1(ab) -> c_to_ri1/1(In1)
